simulink model "demoNPSAUV"  (R2024a)
settings: Solver=ode4  StartTime=0.0  StopTime=100  FixedStep=0.05  RelTol=1e-3  EnableMultiTasking=on
libraries: mssSimulink x3
settings Model: Creator=thor  LastModifiedBy=thor
settings SolverCC: AlgebraicLoopSolver=TrustRegion
settings DataIOCC: LimitDataPoints=on  SaveFormat=Array  SignalLoggingSaveFormat=ModelDataLogs  ReturnWorkspaceOutputs=off  SignalLoggingName=sigsOut
settings OptimizationCC: BooleanDataType=off  InitFltsAndDblsToZero=on  LifeSpan=inf
settings DebuggingCC: SaveWithParameterizedLinksMsg=none  UnderspecifiedInitializationDetection=Classic  MergeDetectMultiDrivingBlocksExec=none  SignalResolutionControl=TryResolveAllWithWarning  MultiTaskDSMMsg=warning  MultiTaskCondExecSysMsg=none  FcnCallInpInsideContextMsg=warning  UnconnectedInputMsg=warning  UnconnectedOutputMsg=warning  UnconnectedLineMsg=warning  SFUnexpectedBacktrackingDiag=warning  SFNoUnconditionalDefaultTransitionDiag=warning  SFExecutionAtInitializationDiag=none  ArithmeticOperatorsInVariantConditions=warning
settings HardwareCC: ProdBitPerPointer=32  ProdBitPerSizeT=32  ProdBitPerPtrDiffT=32  ProdLargestAtomicFloat=None  ProdIntDivRoundTo=Undefined  ProdEndianess=Unspecified  ProdWordSize=32  ProdHWDeviceType=32-bit Generic  TargetUnknown=on
settings ModelReferenceCC: EnableRefExpFcnMdlSchedulingChecks=on  PropagateSignalLabelsOutOfModel=off
settings RTWCC: GPUComputeCapability=3.5  DLArmComputeVersion=19.05
settings CodeAppCC: StateflowObjectComments=on
settings GRTTargetCC: TargetFcnLib=ansi_tfl_tmw.mat  TargetLangStandard=C89/C90 (ANSI)  ModelReferenceCompliant=off  CombineOutputUpdateFcns=off  MatFileLogging=off  GRTInterface=on
settings ConfigComp: CovMetricSettings=dw  CovSaveCumulativeToWorkspaceVar=on  CovSaveSingleToWorkspaceVar=on

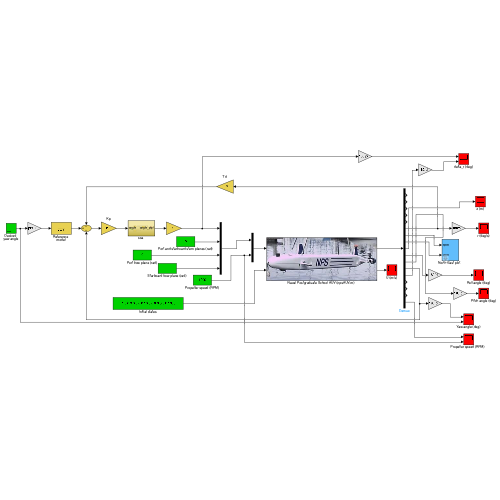
[thumbnail: Simulink's stored preview of the top-level diagram]
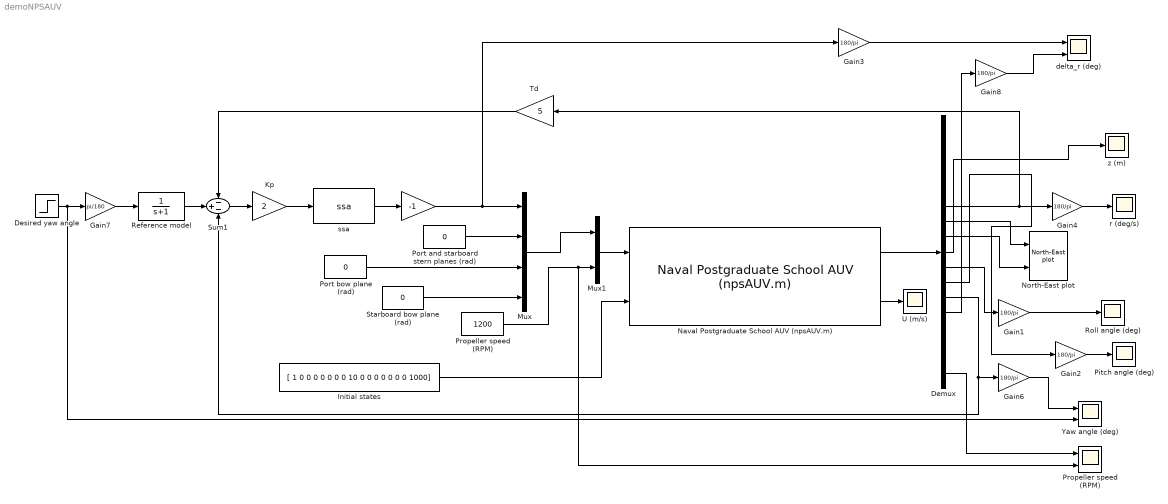
== system demoNPSAUV ==
  "   " : Gain  Gain=-1  SaturateOnIntegerOverflow=on  OutDataTypeStr=Inherit: Same as input  ParamDataTypeStr=Inherit: Same as input
  Demux : Demux  Outputs=17
  Desired yaw angle : Step  Time=10  After=10  SampleTime=0
  Gain{1..4,6,8} (6 alike) : Gain  Gain=180/pi
  Gain7 : Gain  Gain=pi/180
  Initial states : Constant  Value=[ 1 0 0 0 0 0 0 0 10 0 0 0 0 0 0 0 1000]
  Kp : Gain  Gain=2  SaturateOnIntegerOverflow=on  OutDataTypeStr=Inherit: Same as input  ParamDataTypeStr=Inherit: Same as input
  Mux : Mux
  Mux1 : Mux  Inputs=2
  "Naval Postgraduate School AUV (npsAUV.m) " : mssSimulink/Marine craft models/Naval Postgraduate School AUV (npsAUV.m)  SystemSampleTime=-1  VariantActivationTime=update diagram  AllowFlexibleInterface=on  Latency=0  AutoFrameSizeCalculation=off
  "North-East plot  " : mssSimulink/Utilities/Visualization/North-East plot    decimation=100
  Pitch angle (deg) : Scope
  Port and starboard stern planes (rad) : Constant  Value=0
  Port bow plane (rad) : Constant  Value=0
  Propeller speed (RPM) : Constant  Value=1200
  "Propeller speed (RPM)  " : Scope  NumInputPorts=2
  Reference model : TransferFcn  Denominator=[1 1]
  Roll angle (deg) : Scope
  Starboard bow plane (rad) : Constant  Value=0
  Sum1 : Sum  Inputs=-+-  InputSameDT=on  SaturateOnIntegerOverflow=on  OutDataTypeStr=Inherit: Same as first input
  Td : Gain  Gain=5  SaturateOnIntegerOverflow=on  OutDataTypeStr=Inherit: Same as input  ParamDataTypeStr=Inherit: Same as input
  U (m/s) : Scope
  Yaw angle (deg) : Scope  NumInputPorts=2
  delta_r (deg) : Scope  NumInputPorts=2
  r (deg/s) : Scope
  "ssa " : mssSimulink/Utilities/Math Operations/ssa  SystemSampleTime=-1  VariantActivationTime=update diagram  AllowFlexibleInterface=on  Latency=0  AutoFrameSizeCalculation=off
  z (m) : Scope
  wires:
  Sum1/1 -> Kp/1
  Td/1 -> Sum1/1
  Initial states/1 -> "Naval Postgraduate School AUV (npsAUV.m) "/2
  Propeller speed (RPM)/1 -> "Propeller speed (RPM)  "/2, Mux1/2
  Port and starboard stern planes (rad)/1 -> Mux/2
  Port bow plane (rad)/1 -> Mux/3
  Starboard bow plane (rad)/1 -> Mux/4
  "Naval Postgraduate School AUV (npsAUV.m) "/1 -> Demux/1
  Demux/6 -> Gain4/1, Td/1
  Demux/7 -> "North-East plot  "/1
  Demux/9 -> z (m)/1
  Demux/10 -> Gain1/1
  Demux/11 -> Gain2/1
  "Naval Postgraduate School AUV (npsAUV.m) "/2 -> U (m/s)/1
  Mux1/1 -> "Naval Postgraduate School AUV (npsAUV.m) "/1
  Gain2/1 -> Pitch angle (deg)/1
  Gain1/1 -> Roll angle (deg)/1
  Reference model/1 -> Sum1/2
  Mux/1 -> Mux1/1
  Demux/12 -> Sum1/3, Gain6/1
  Gain6/1 -> Yaw angle (deg)/1
  Gain3/1 -> delta_r (deg)/1
  Gain4/1 -> r (deg/s)/1
  Gain7/1 -> Reference model/1
  "   "/1 -> Gain3/1, Mux/1
  Desired yaw angle/1 -> Yaw angle (deg)/2, Gain7/1
  Kp/1 -> "ssa "/1
  "ssa "/1 -> "   "/1
  Demux/8 -> "North-East plot  "/2
  Demux/17 -> "Propeller speed (RPM)  "/1
  Demux/13 -> Gain8/1
  Gain8/1 -> delta_r (deg)/2
